simulink subsystem "Subsys_GFormConv_OuterCtrl_Droop"  (R2022b)
settings: Solver=VariableStepAuto  StartTime=0.0  StopTime=10.0  RelTol=1e-3
model mask{f_n=50, s_droop_Pf=0.05, s_droop_QV=0.1, T_Q=0.2, T_s_ctrl=1e-3, T_s_PWM_meas=1e-4}
  mask prompts: f_n "Nominal Frequency [Hz]"; s_droop_Pf "Droop constant kP (df[pu]/dP[pu])"; s_droop_QV "Droop constant kQ (dV[pu]/dQ[pu])"; T_Q "PT1 time constant QV-loop T_Q [s]"; T_s_ctrl "Controller sample time [s]"; T_s_PWM_meas "PWM and measurements sample time [s]"
undefined symbols (not defined in the file): alpha_LPF_Q
libraries: simulink x1
settings Model: Creator=winkens  LastModifiedBy=winkens
settings SolverCC: AlgebraicLoopSolver=TrustRegion
settings DebuggingCC: UnconnectedInputMsg=warning  UnconnectedOutputMsg=warning  UnconnectedLineMsg=warning  SFMachineParentedDataDiag=warning
settings ModelReferenceCC: EnableRefExpFcnMdlSchedulingChecks=on
settings RTWCC: DLArmComputeVersion=19.05

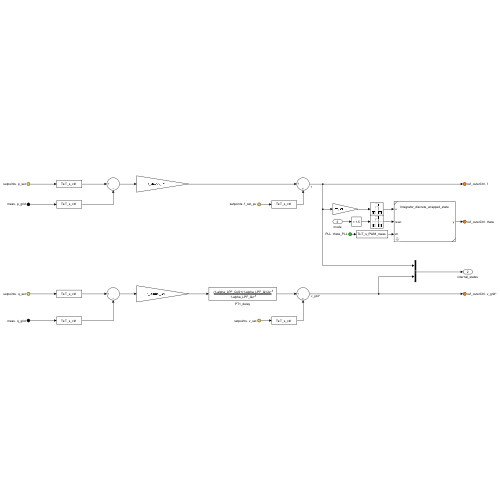
[thumbnail: Simulink's stored preview of the top-level diagram]
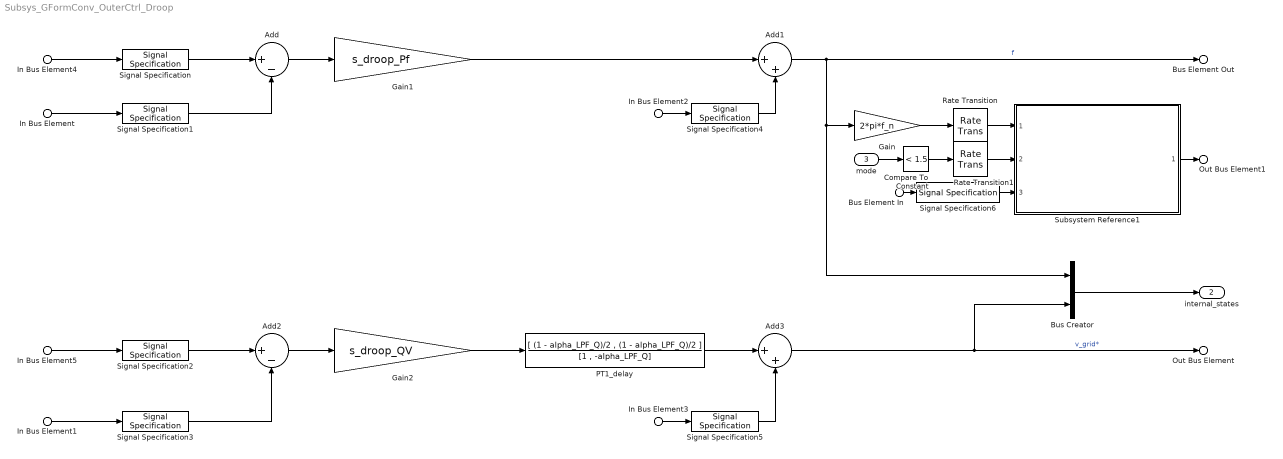
== system Subsys_GFormConv_OuterCtrl_Droop ==
  In Bus Element : Inport  PortName=meas  Element=p_grid
  In Bus Element1 : Inport  PortName=meas  Element=q_grid
  In Bus Element2 : Inport  Port=2  PortName=setpoints  Element=f_set_pu
  In Bus Element3 : Inport  Port=2  PortName=setpoints  Element=v_set
  In Bus Element4 : Inport  Port=2  PortName=setpoints  Element=p_set
  In Bus Element5 : Inport  Port=2  PortName=setpoints  Element=q_set
  mode : Inport  Port=3
  Bus Element In : Inport  Port=4  PortName=PLL  Element=theta_PLL
  Add : Sum  Inputs=|+-
  Add1 : Sum  Inputs=|++
  Add2 : Sum  Inputs=|+-
  Add3 : Sum  Inputs=|++
  Bus Creator : BusCreator  Inputs=2
  Compare To Constant : simulink/Logic and Bit Operations/Compare To Constant  relop=<  const=1.5  OutDataTypeStr=boolean
  Gain : Gain  Gain=2*pi*f_n
  Gain1 : Gain  Gain=s_droop_Pf
  Gain2 : Gain  Gain=s_droop_QV
  PT1_delay : DiscreteFilter  Numerator=[ (1 - alpha_LPF_Q)/2 , (1 - alpha_LPF_Q)/2 ]  Denominator=[1 , -alpha_LPF_Q]  SampleTime=T_s_ctrl
  Rate Transition : RateTransition  Deterministic=off  OutPortSampleTime=T_s_PWM_meas
  Rate Transition1 : RateTransition  Deterministic=off  OutPortSampleTime=T_s_PWM_meas
  Signal Specification{,1..5} (6 alike) : SignalSpecification  SampleTime=T_s_ctrl
  Signal Specification6 : SignalSpecification  SampleTime=T_s_PWM_meas
  Subsystem Reference1 : Subsystem  ReferencedSubsystem=Integrator_discrete_wrapped_state  WrappedStateUpperValue=2*pi  WrappedStateLowerValue=0  x_0=0  T_s=T_s_PWM_meas
  Out Bus Element1 : Outport  PortName=ref_outerCtrl  Element=theta
  Bus Element Out : Outport  PortName=ref_outerCtrl  Element=f
  Out Bus Element : Outport  PortName=ref_outerCtrl  Element=v_grid*
  internal_states : Outport  Port=2
  wires:
  Add2/1 -> Gain2/1
  Gain2/1 -> PT1_delay/1
  PT1_delay/1 -> Add3/1
  Add1/1 -> Bus Element Out/1, Gain/1, Bus Creator/1  "f"
  Add/1 -> Gain1/1
  Gain1/1 -> Add1/1
  In Bus Element/1 -> Signal Specification1/1
  Bus Creator/1 -> internal_states/1
  Add3/1 -> Bus Creator/2, Out Bus Element/1  "v_grid*"
  In Bus Element1/1 -> Signal Specification3/1
  In Bus Element4/1 -> Signal Specification/1
  In Bus Element2/1 -> Signal Specification4/1
  In Bus Element5/1 -> Signal Specification2/1
  In Bus Element3/1 -> Signal Specification5/1
  Bus Element In/1 -> Signal Specification6/1
  Compare To Constant/1 -> Rate Transition1/1
  mode/1 -> Compare To Constant/1
  Gain/1 -> Rate Transition/1
  Subsystem Reference1/1 -> Out Bus Element1/1
  Signal Specification/1 -> Add/1
  Signal Specification1/1 -> Add/2
  Signal Specification2/1 -> Add2/1
  Signal Specification3/1 -> Add2/2
  Signal Specification4/1 -> Add1/2
  Signal Specification5/1 -> Add3/2
  Signal Specification6/1 -> Subsystem Reference1/3
  Rate Transition/1 -> Subsystem Reference1/1
  Rate Transition1/1 -> Subsystem Reference1/2
